simulink subsystem "servoModel"  (R2026a)
settings: Solver=VariableStepAuto
settings Model: Creator=maxhu  LastModifiedBy=maxhu

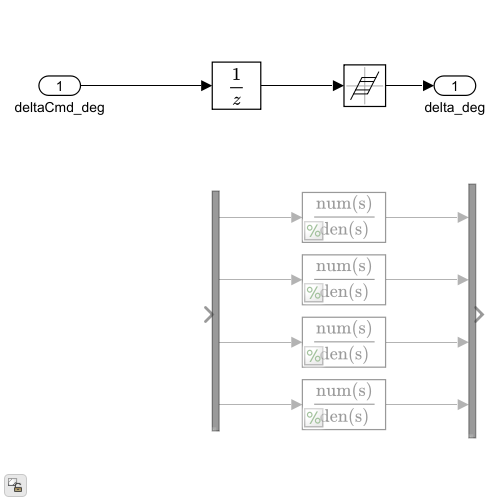
[thumbnail: Simulink's stored preview of the top-level diagram]
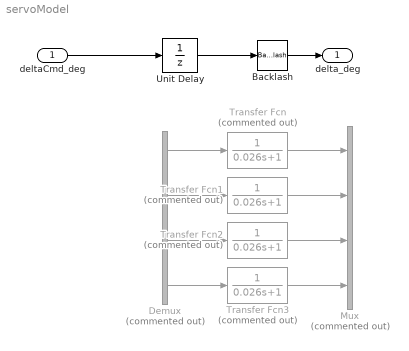
== system servoModel ==
  deltaCmd_deg : Inport
  Backlash : Backlash
  Demux : Demux  Commented=on
  Mux : Mux  Commented=on
  Transfer Fcn{,1..3} (4 alike) : TransferFcn  Commented=on  Denominator=[0.026 1]
  Unit Delay : UnitDelay  SampleTime=-1
  delta_deg : Outport
  wires:
  Unit Delay/1 -> Backlash/1
  deltaCmd_deg/1 -> Unit Delay/1
  Transfer Fcn/1 -> Mux/1
  Demux/1 -> Transfer Fcn/1
  Demux/2 -> Transfer Fcn1/1
  Transfer Fcn1/1 -> Mux/2
  Demux/3 -> Transfer Fcn2/1
  Transfer Fcn2/1 -> Mux/3
  Demux/4 -> Transfer Fcn3/1
  Transfer Fcn3/1 -> Mux/4
  Backlash/1 -> delta_deg/1
